simulink model "DCHR_A41_Closed_Loop"  (R2026a)
settings: Solver=FixedStepDiscrete  StopTime=603900  FixedStep=900
settings Model: Creator=Lysda  LastModifiedBy=Lysda

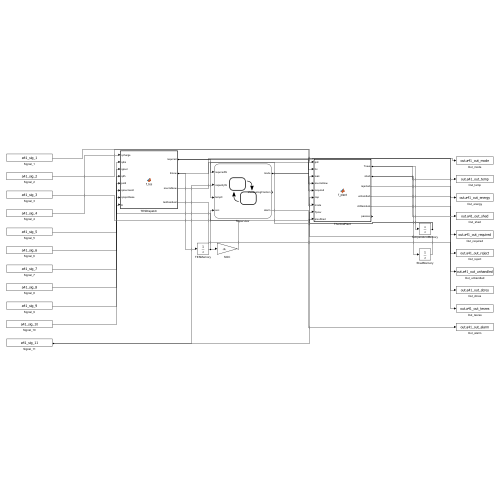
[thumbnail: Simulink's stored preview of the top-level diagram]
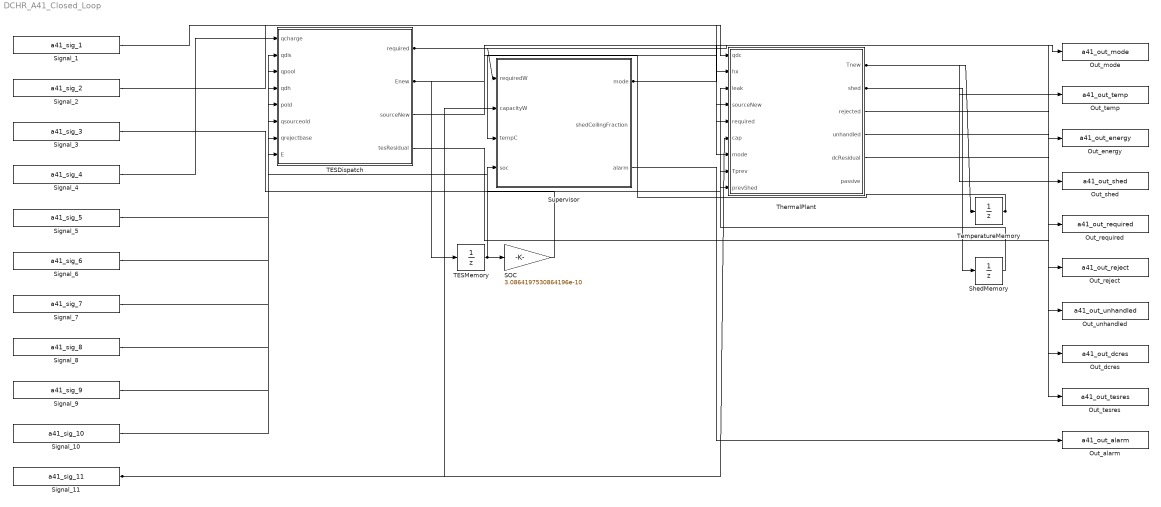
== system DCHR_A41_Closed_Loop ==
  Out_alarm : ToWorkspace  VariableName=a41_out_alarm  SampleTime=-1
  Out_dcres : ToWorkspace  VariableName=a41_out_dcres  SampleTime=-1
  Out_energy : ToWorkspace  VariableName=a41_out_energy  SampleTime=-1
  Out_mode : ToWorkspace  VariableName=a41_out_mode  SampleTime=-1
  Out_reject : ToWorkspace  VariableName=a41_out_reject  SampleTime=-1
  Out_required : ToWorkspace  VariableName=a41_out_required  SampleTime=-1
  Out_shed : ToWorkspace  VariableName=a41_out_shed  SampleTime=-1
  Out_temp : ToWorkspace  VariableName=a41_out_temp  SampleTime=-1
  Out_tesres : ToWorkspace  VariableName=a41_out_tesres  SampleTime=-1
  Out_unhandled : ToWorkspace  VariableName=a41_out_unhandled  SampleTime=-1
  SOC : Gain  Gain=3.0864197530864196e-10
  ShedMemory : UnitDelay  SampleTime=-1
  Signal_1 : FromWorkspace  VariableName=a41_sig_1
  Signal_10 : FromWorkspace  VariableName=a41_sig_10
  Signal_11 : FromWorkspace  VariableName=a41_sig_11
  Signal_2 : FromWorkspace  VariableName=a41_sig_2
  Signal_3 : FromWorkspace  VariableName=a41_sig_3
  Signal_4 : FromWorkspace  VariableName=a41_sig_4
  Signal_5 : FromWorkspace  VariableName=a41_sig_5
  Signal_6 : FromWorkspace  VariableName=a41_sig_6
  Signal_7 : FromWorkspace  VariableName=a41_sig_7
  Signal_8 : FromWorkspace  VariableName=a41_sig_8
  Signal_9 : FromWorkspace  VariableName=a41_sig_9
  Supervisor : Stateflow chart  TreatAsAtomicUnit=on
  TESDispatch : MATLAB Function  TreatAsAtomicUnit=on
  TESMemory : UnitDelay  InitialCondition=1620000000  SampleTime=-1
  TemperatureMemory : UnitDelay  InitialCondition=30  SampleTime=-1
  ThermalPlant : MATLAB Function  TreatAsAtomicUnit=on
  wires:
  TESMemory/1 -> SOC/1, TESDispatch/8(E)
  SOC/1 -> Supervisor/4(soc)
  TemperatureMemory/1 -> Supervisor/3(tempC), ThermalPlant/8(Tprev)
  TESDispatch/1(required) -> Supervisor/1(requiredW), ThermalPlant/5(required), Out_required/1
  TESDispatch/2(Enew) -> TESMemory/1, Out_energy/1
  ThermalPlant/1(Tnew) -> TemperatureMemory/1, Out_temp/1
  ThermalPlant/2(shed) -> ShedMemory/1, Out_shed/1
  Signal_4/1 -> TESDispatch/1(qcharge)
  Signal_5/1 -> TESDispatch/2(qdis)
  Signal_6/1 -> TESDispatch/3(qpool)
  Signal_7/1 -> TESDispatch/4(qdh)
  Signal_8/1 -> TESDispatch/5(pold)
  Signal_9/1 -> TESDispatch/6(qsourceold)
  Signal_10/1 -> TESDispatch/7(qrejectbase)
  Signal_1/1 -> ThermalPlant/1(qdc)
  Signal_2/1 -> ThermalPlant/2(hx)
  Signal_3/1 -> ThermalPlant/3(leak)
  TESDispatch/3(sourceNew) -> ThermalPlant/4(sourceNew)
  Signal_11/1 -> Supervisor/2(capacityW), ThermalPlant/6(cap)
  Supervisor/1(mode) -> ThermalPlant/7(mode), Out_mode/1
  ShedMemory/1 -> ThermalPlant/9(prevShed)
  ThermalPlant/3(rejected) -> Out_reject/1
  ThermalPlant/4(unhandled) -> Out_unhandled/1
  ThermalPlant/5(dcResidual) -> Out_dcres/1
  TESDispatch/4(tesResidual) -> Out_tesres/1
  Supervisor/3(alarm) -> Out_alarm/1

== matlab function DCHR_A41_Closed_Loop/ThermalPlant ==
  data: qdc input; Tnew output; hx input; leak input; sourceNew input; required input; cap input; mode input; Tprev input; prevShed input; shed output; rejected output; unhandled output; dcResidual output; passive output
function [Tnew,shed,rejected,unhandled,dcResidual,passive] = f_plant(qdc,hx,leak,sourceNew,required,cap,mode,Tprev,prevShed)
%#codegen
dt=900;
if mode==1 || mode==2
    ceiling=.4;
else
    ceiling=0;
end
target=min([max(0,required-cap),ceiling*qdc,required]);
if ceiling>0
    shed=min(target,min(prevShed,qdc)+15000);
else
    shed=0;
end
rejected=min(required-shed,cap);
unhandled=max(0,required-shed-rejected);
passive=2000*max(0,Tprev-30);
Tnew=max(30,Tprev+dt*(unhandled-passive)/8e6);
dcResidual=qdc-shed-hx-sourceNew-leak-rejected-unhandled;

== matlab function DCHR_A41_Closed_Loop/TESDispatch ==
  data: qcharge input; required output; qdis input; qpool input; qdh input; pold input; qsourceold input; qrejectbase input; E input; Enew output; sourceNew output; tesResidual output
function [required,Enew,sourceNew,tesResidual] = f_tes(qcharge,qdis,qpool,qdh,pold,qsourceold,qrejectbase,E)
%#codegen
dt=900; Emax=900*3.6e6;
loss=.002*E/86400;
room=max(0,(Emax-E+dt*(qdis/.91+loss))/(dt*.93));
charge=min(qcharge,room);
Enew=max(0,min(Emax,E+dt*(.93*charge-qdis/.91-loss)));
oldCond=qpool+qdh+qcharge;
newCond=oldCond-(qcharge-charge);
if oldCond>1e-8
    newPower=pold*newCond/oldCond;
else
    newPower=0;
end
sourceNew=newCond-newPower;
required=max(0,qrejectbase+qsourceold-sourceNew);
tesResidual=Enew-E-dt*(.93*charge-qdis/.91-loss);

== stateflow chart DCHR_A41_Closed_Loop/Supervisor ==
  state NORMAL
    entry: mode=0; shedCeilingFraction=0; alarm=0;
  state DEGRADED
    entry: mode=1; shedCeilingFraction=0.4; alarm=1;
  state TES_FULL
    entry: mode=3; shedCeilingFraction=0; alarm=1;
  state CRITICAL
    entry: mode=2; shedCeilingFraction=0.4; alarm=2;
  DEGRADED -> NORMAL [order 2] : [requiredW + 5000 <= capacityW && tempC < 39 && soc < 0.999]
  (default) -> NORMAL
  TES_FULL -> NORMAL [order 1] : [soc <= 0.98 && requiredW + 5000 <= capacityW && tempC < 39]
  DEGRADED -> TES_FULL [order 3] : [soc >= 0.999 && requiredW + 5000 <= capacityW && tempC < 39]
  TES_FULL -> DEGRADED [order 2] : [requiredW > capacityW + 1e-6 && tempC < 42 && capacityW > 0]
  NORMAL -> DEGRADED [order 1] : [requiredW > capacityW + 1e-6 && tempC < 42 && capacityW > 0]
  CRITICAL -> DEGRADED : [tempC < 39 && capacityW > 0]
  NORMAL -> CRITICAL [order 2] : [tempC >= 42 || capacityW <= 0]
  NORMAL -> TES_FULL [order 3] : [soc >= 0.999 && requiredW <= capacityW && tempC < 42 && capacityW > 0]
  DEGRADED -> CRITICAL [order 1] : [tempC >= 42 || capacityW <= 0]
  TES_FULL -> CRITICAL [order 3] : [tempC >= 42 || capacityW <= 0]
  data: requiredW input; capacityW input; tempC input; soc input; mode output; shedCeilingFraction output; alarm output
